simulink model "inversed"  (R2023b)
settings: Solver=VariableStepAuto  StartTime=0.0  StopTime=10  MaxStep=0.05  RelTol=1e-3
values from neighbouring files (symbols this model uses):
  i = m*l^2    [mask123.m]    (also in mask2.m)
libraries: simulink_extras x2, slpidlib x1
settings Model: Creator=macbook  LastModifiedBy=macbook
settings DataIOCC: ReturnWorkspaceOutputs=off

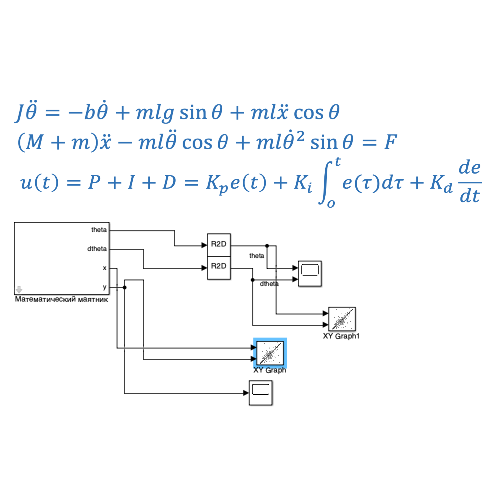
[thumbnail: Simulink's stored preview of the top-level diagram]
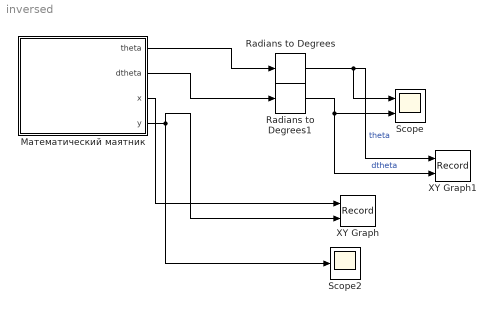
== system inversed ==
  Radians to Degrees : simulink_extras/Transformations/Radians to Degrees
  Radians to Degrees1 : simulink_extras/Transformations/Radians to Degrees
  Scope : Scope  NumInputPorts=2
  Scope2 : Scope
  XY Graph : Record  FileSettingsInternal="{\"entries\":[{\"content\":{\"excelSettings\":{\"content\":{},\"type\":\"Streamout.ExcelSettings\"}},\"type\":\"Streamout.FileSettingStorage\",\"uuid\":\"\"}],\"packageUris\":[\"http:\\/\\/schema.mathworks.com\\/mf0\\/streamout_blocks\\/R2020a\"],\"version\":\"1.0\"}"  Layout=[1 1]  SignalsInternal="{\"entries\":[{\"content\":{\"signals\":[{\"content\":{\"blockPath\":[],\"dimensions\":[1],\"domain\":\"\",\"lineColor\":\"#a2142f\",\"plots\":[1],\"port\":1,\"sid\":[\"\"],\"signalID\":7404,\"signalName\":\"Математический маятник:3\"},\"type\":\"RecordBlkView.Signal\",\"uuid\":\"\"},{\"content\":{\"blockPath\":[],\"dimensions\":[1],\"domain\":\"\",\"lineColor\":\"#139fff\",\"plots\":[1],\"port\":2,\"sid\":[\"\"],\"signalID\":7408,\"signalName\":\"Математический маятник:4\"},\"type\":\"RecordBlkView.Signal\",\"uuid\":\"\"}]},\"type\":\"RecordBlkView.InputSignals\",\"uuid\":\"\"}],\"packageUris\":[\"http:\\/\\/schema.mathworks.com\\/mf0\\/streamout_blocks\\/R2020a\"],\"version\":\"1.0\"}"  VisualizationBindings="{\"xyplotplugin\":{\"info\":[{\"series\":[{\"bindingParametersList\":[{\"parameter\":\"X-Axis\",\"signalID\":7404,\"signalName\":\"Математический маятник:3\"},{\"parameter\":\"Y-Axis\",\"signalID\":7408,\"signalName\":\"Математический маятник:4\"}],\"seriesID\":27144}],\"subplotID\":1}]}}"  CompatibilityTag=XY
  XY Graph1 : Record  FileSettingsInternal="{\"entries\":[{\"content\":{\"excelSettings\":{\"content\":{},\"type\":\"Streamout.ExcelSettings\"}},\"type\":\"Streamout.FileSettingStorage\",\"uuid\":\"\"}],\"packageUris\":[\"http:\\/\\/schema.mathworks.com\\/mf0\\/streamout_blocks\\/R2020a\"],\"version\":\"1.0\"}"  Layout=[1 1]  SignalsInternal="{\"entries\":[{\"content\":{\"signals\":[{\"content\":{\"blockPath\":[],\"dimensions\":[1],\"domain\":\"\",\"lineColor\":\"#a2142f\",\"plots\":[1],\"port\":1,\"sid\":[\"\"],\"signalID\":7412,\"signalName\":\"theta\"},\"type\":\"RecordBlkView.Signal\",\"uuid\":\"\"},{\"content\":{\"blockPath\":[],\"dimensions\":[1],\"domain\":\"\",\"lineColor\":\"#139fff\",\"plots\":[1],\"port\":2,\"sid\":[\"\"],\"signalID\":7416,\"signalName\":\"dtheta\"},\"type\":\"RecordBlkView.Signal\",\"uuid\":\"\"}]},\"type\":\"RecordBlkView.InputSignals\",\"uuid\":\"\"}],\"packageUris\":[\"http:\\/\\/schema.mathworks.com\\/mf0\\/streamout_blocks\\/R2020a\"],\"version\":\"1.0\"}"  VisualizationBindings="{\"xyplotplugin\":{\"info\":[{\"series\":[{\"bindingParametersList\":[{\"parameter\":\"X-Axis\",\"signalID\":7412,\"signalName\":\"theta\"},{\"parameter\":\"Y-Axis\",\"signalID\":7416,\"signalName\":\"dtheta\"}],\"seriesID\":30809}],\"subplotID\":1}]}}"  CompatibilityTag=XY
  Математический маятник : Subsystem  mask{m=1, l=1, b=0, g=9.81, angel=5, Mas=1, F=0}
      mask prompts: m "Масса"; l "Длина"; angel "Начальный угол"; Mas "M"
  wires:
  Математический маятник/1(theta) -> Radians to Degrees/1
  Математический маятник/2(dtheta) -> Radians to Degrees1/1
  Radians to Degrees/1 -> XY Graph1/1, Scope/1  "theta"
  Radians to Degrees1/1 -> XY Graph1/2, Scope/2  "dtheta"
  Математический маятник/3(x) -> XY Graph/1
  Математический маятник/4(y) -> XY Graph/2, Scope2/1

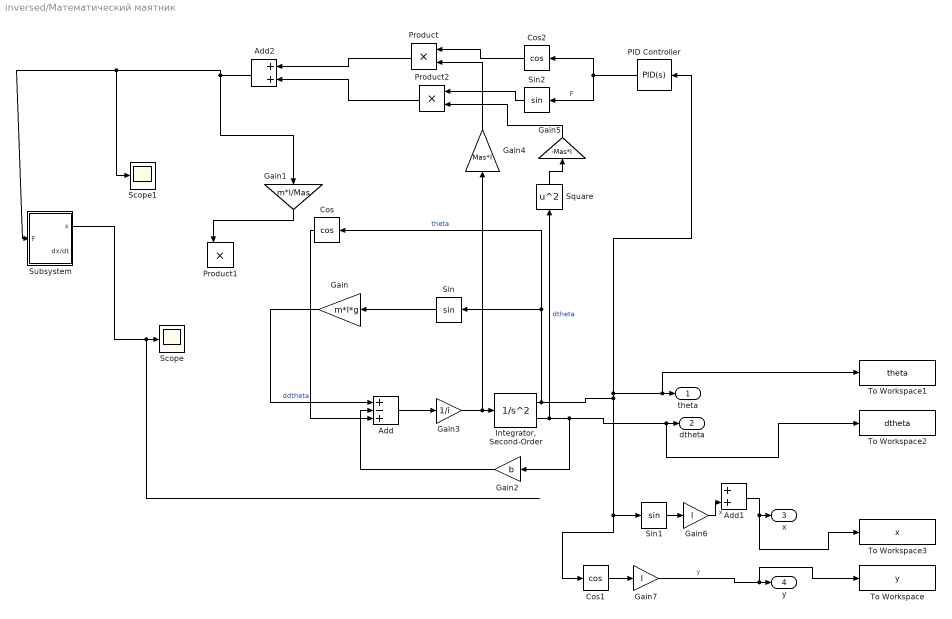
== system inversed/Математический маятник ==
  Add : Sum  Inputs=+-+
  Add1 : Sum
  Add2 : Sum
  Cos : Trigonometry  Operator=cos
  Cos1 : Trigonometry  Operator=cos
  Cos2 : Trigonometry  Operator=cos
  Gain : Gain  Gain=m*l*g
  Gain1 : Gain  Gain=m*l/Mas
  Gain2 : Gain  Gain=b
  Gain3 : Gain  Gain=1/i
  Gain4 : Gain  Gain=Mas*l
  Gain5 : Gain  Gain=-Mas*l
  Gain6 : Gain  Gain=l
  Gain7 : Gain  Gain=l
  "Integrator, Second-Order" : SecondOrderIntegrator  ICX=deg2rad(angel)  ICDXDT=0
  PID Controller : slpidlib/PID Controller  Controller=PID  Form=Parallel  TimeDomain=Continuous-time  UseExternalTs=off  SampleTime=-1  IntegratorMethod=Forward Euler  FilterMethod=Forward Euler  ControllerParametersSource=internal  P=0  I=0  UseKiTs=off  D=0  N=100  UseFilter=on  TunerSelectOption=Transfer Function Based (PID Tuner App)  InitialConditionSource=internal  InitialConditionForIntegrator=0  InitialConditionForFilter=0  DifferentiatorICPrevScaledInput=0  ExternalReset=none  TrackingMode=off  Kt=1  LimitOutput=off  SatLimitsSource=internal  UpperSaturationLimit=inf  LowerSaturationLimit=-inf  LinearizeAsGain=on  AntiWindupMode=none  Kb=1  LimitIntegrator=off  UpperIntegratorSaturationLimit=inf  LowerIntegratorSaturationLimit=-inf  POutMin=[]  POutMax=[]  IOutMin=[]  IOutMax=[]  DOutMin=[]  DOutMax=[]  NOutMin=[]  NOutMax=[]  SumOutMin=[]  SumOutMax=[]  SaturationOutMin=[]  SaturationOutMax=[]  PParamMin=[]  PParamMax=[]  IParamMin=[]  IParamMax=[]  DParamMin=[]  DParamMax=[]  NParamMin=[]  NParamMax=[]  KbParamMin=[]  KbParamMax=[]  KtParamMin=[]  KtParamMax=[]  KbOutMin=[]  KbOutMax=[]  KtOutMin=[]  KtOutMax=[]  IntegratorOutMin=[]  IntegratorOutMax=[]  FilterOutMin=[]  FilterOutMax=[]  SumI1OutMin=[]  SumI1OutMax=[]  SumI2OutMin=[]  SumI2OutMax=[]  SumI3OutMin=[]  SumI3OutMax=[]  SumI4OutMin=[]  SumI4OutMax=[]  SumDOutMin=[]  SumDOutMax=[]  DifferentiatorOutMin=[]  DifferentiatorOutMax=[]  FilterDiffOutCoefMin=[]  FilterDiffOutCoefMax=[]  ReciprocalOutMin=[]  ReciprocalOutMax=[]  SumDenOutMin=[]  SumDenOutMax=[]  SumNumOutMin=[]  SumNumOutMax=[]  DivideOutMin=[]  DivideOutMax=[]  UdiffTsProdOutMin=[]  UdiffTsProdOutMax=[]  NTsProdOutMin=[]  NTsProdOutMax=[]  UintegralTsProdOutMin=[]  UintegralTsProdOutMax=[]  UngainTsProdOutMin=[]  UngainTsProdOutMax=[]  ClampingZeroOutDataTypeStr=Inherit: Inherit via back propagation  ClampingZeroOutMin=[]  ClampingZeroOutMax=[]  FilterDenConstantOutDataTypeStr=Inherit: Inherit via back propagation  FilterDenConstantOutMin=[]  FilterDenConstantOutMax=[]  PCopyOutDataTypeStr=Inherit: Inherit via back propagation  PCopyOutMin=[]  PCopyOutMax=[]  NCopyOutDataTypeStr=Inherit: Inherit via back propagation  NCopyOutMin=[]  NCopyOutMax=[]  IntegratorContinuousStateAttributes=''  IntegratorStateMustResolveToSignalObject=off  IntegratorRTWStateStorageClass=Auto  FilterContinuousStateAttributes=''  FilterStateMustResolveToSignalObject=off  FilterRTWStateStorageClass=Auto  ParallelPVariant=InternalParameters  IdealPVariant=Disabled  IVariant=InternalParameters  DVariant=InternalParameters  IntegratorVariant=Continuous  SatVariant=Disabled  AWVariant=Passthrough  PCopyVariant=Disabled  TRVariant=Disabled  FdbkBlocksVariant=Forward  IdealPFdbkVariant=Disabled  SatFdbkVariant=Disabled  DerivativeFilterVariant=ContFilter  NVariant=InternalParameters  NCopyVariant=Disabled  FilterICVariant=InternalICsFilter  IntegratorICVariant=InternalICs  ExternalResetVariant=Disabled  TRSumVariant=Passthrough  SumFdbkVariant=Disabled  SumVariant=Sum_PID  TsampFilterVariant=InternalTs  TsampNgainVariant=Passthrough  TsampIntegralVariant=Disabled_SignalSpec  ExternalSaturationOutDataTypeStr=Inherit: Same as second input
  Product : Product
  Product1 : Product
  Product2 : Product
  Scope : Scope
  Scope1 : Scope
  Sin : Trigonometry
  Sin1 : Trigonometry
  Sin2 : Trigonometry
  Square : Math  Operator=square
  Subsystem : Subsystem
  To Workspace : ToWorkspace  VariableName=y  SampleTime=-1
      settings: Save2DSignal=2-D array (concatenate along first dimension)
  To Workspace1 : ToWorkspace  VariableName=theta  SampleTime=-1
      settings: Save2DSignal=2-D array (concatenate along first dimension)
  To Workspace2 : ToWorkspace  VariableName=dtheta  SampleTime=-1
      settings: Save2DSignal=2-D array (concatenate along first dimension)
  To Workspace3 : ToWorkspace  VariableName=x  SampleTime=-1
      settings: Save2DSignal=2-D array (concatenate along first dimension)
  theta : Outport
  dtheta : Outport  Port=2
  x : Outport  Port=3
  y : Outport  Port=4
  wires:
  "Integrator, Second-Order"/2 -> To Workspace2/1, dtheta/1, Gain2/1, Square/1  "dtheta"
  "Integrator, Second-Order"/1 -> Cos/1, Sin/1, To Workspace1/1, theta/1, PID Controller/1, Cos1/1, Sin1/1  "theta"
  Gain/1 -> Add/1  "ddtheta"
  Add/1 -> Gain3/1
  Gain2/1 -> Add/2
  Sin1/1 -> Gain6/1
  Cos1/1 -> Gain7/1
  Gain7/1 -> To Workspace/1, y/1  "y"
  Sin/1 -> Gain/1
  Subsystem/1(x) -> Scope/1
  Gain6/1 -> Add1/2  "x"
  Add1/1 -> To Workspace3/1, x/1
  Gain1/1 -> Product1/1
  Cos/1 -> Add/3
  Gain3/1 -> Gain4/1, "Integrator, Second-Order"/1
  PID Controller/1 -> Sin2/1, Cos2/1  "F"
  Cos2/1 -> Product/1
  Gain4/1 -> Product/2
  Square/1 -> Gain5/1
  Gain5/1 -> Product2/2
  Sin2/1 -> Product2/1
  Product/1 -> Add2/1
  Product2/1 -> Add2/2
  Add2/1 -> Scope1/1, Subsystem/1(F), Gain1/1

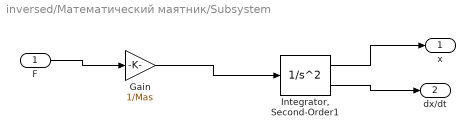
== system inversed/Математический маятник/Subsystem ==
  F : Inport
  Gain : Gain  Gain=1/Mas
  "Integrator, Second-Order1" : SecondOrderIntegrator
  x : Outport
  dx/dt : Outport  Port=2
  wires:
  Gain/1 -> "Integrator, Second-Order1"/1
  "Integrator, Second-Order1"/2 -> dx/dt/1
  "Integrator, Second-Order1"/1 -> x/1
  F/1 -> Gain/1
